simulink model "single_phase_ttype_inverter"  (R2026a)
settings: Solver=ode23tb  StopTime=simlength  FixedStep=tc  MaxStep=glb_time.tc
values from neighbouring files (symbols this model uses):
  afe_ctrl = param.afe.ctrl    [init_model.m]
  afe_pwm_phase_shift_mod1 = param.afe.behav.pwm_phase_shift_mod1    [init_model.m]
  DThs_init = param.thermal.DThs_init    [init_model.m]
  filters = param.ctrl.filters    [init_model.m]
  frt_data = param.frt.data    [init_model.m]
  glb_time = param.glb_time    [init_model.m]
  grid_emu = param.grid.emu    [init_model.m]
  kepsilon = param.spinv.kepsilon    [init_model.m]
  kp_align = param.ctrl.kp_align    [init_model.m]
  lim_down_align = param.ctrl.lim_down_align    [init_model.m]
  lim_up_align = param.ctrl.lim_up_align    [init_model.m]
  mavarage_filter_frequency_base_order = param.ctrl.mavarage_filter_frequency_base_order    [init_model.m]
  omega_set = param.spinv.omega_set    [init_model.m]
  single_phase_inverter_ctrl = param.spinv.ctrl    [init_model.m]
  Tambient = param.thermal.Tambient    [init_model.m]
  time_aux_power_supply_fault = param.sim.time_aux_power_supply_fault    [init_model.m]
  time_step_ref_1 = param.spinv.ref.time_step_ref_1    [init_model.m]
  time_step_ref_2 = param.spinv.ref.time_step_ref_2    [init_model.m]
  time_step_ref_3 = param.spinv.ref.time_step_ref_3    [init_model.m]
undefined symbols (not defined in the file or in its folder): delta_fht1, hwdata, ki_align, Ld_fht1, magnitude, omega_fht1, ts_inv, Vac_FS, Vdc_nom, Xbez
libraries: fl_lib x61, nesl_utility x39, moving_average_filter x11, moving_average_filter_cc x8, discrete_time_low_pass_filter x4, sl_discontinuities x3, single_phase_transformer_lib x3, linear_double_integrator_observer_ccaller x2, phase_shift_filter_ccaller x2, threephase_inductor_lib x1, dclink_for_two_levels x1, three_phase_pwm_modulator x1
(part 5 of 9)

== system single_phase_ttype_inverter/single_phase_inverter/single phase inverter control/single_phase_inverter_ctrl/single_phase_current_control/current_reference_generation ==
  mag_ref : Inport
  phase : Inport  Port=2
  Bus Creator : BusCreator  Inputs=2
  Product : Product
  Product1 : Product
  Sin : Trigonometry  Operator=cos
  Sin1 : Trigonometry
  is_ref : Outport
  id_ref : Outport  Port=2
  wires:
  Sin/1 -> Product/2
  phase/1 -> Sin1/1, Sin/1
  mag_ref/1 -> id_ref/1, Product1/1, Product/1
  Sin1/1 -> Product1/2
  Product/1 -> Bus Creator/1  "is_ref_alpha"
  Product1/1 -> Bus Creator/2  "is_ref_beta"
  Bus Creator/1 -> is_ref/1

== system single_phase_ttype_inverter/single_phase_inverter/single phase inverter control/single_phase_inverter_ctrl/single_phase_current_control/dqpi_current_controller ==
  id_ref : Inport
  Bus Creator : BusCreator  Inputs=3
  Bus Creator1 : BusCreator  Inputs=3
  Constant : Constant
  Variant Source : VariantSource  VariantControls={use_current_controller_from_ccaller_mod1 == 0, use_current_controller_from_ccaller_mod1 == 1}
  Variant Source1 : VariantSource  VariantControls={use_current_controller_from_ccaller_mod1 == 0, use_current_controller_from_ccaller_mod1 == 1}
  alphabeta2dq : Subsystem
  dq2alphabeta : Subsystem
  dq_vector_pi : Subsystem
  dq_vector_pi_ccaller : Subsystem
  dq_vector_pi_tracking : Scope  NumInputPorts=2
      settings: ActiveDisplayYMinimum=-0.073650141288039941  ActiveDisplayYMaximum=0.19925097179955883  DataLoggingVariableName=ScopeData8
  i2alphabeta : Subsystem
  virtual_alpha_beta_currents : Scope  NumInputPorts=3
      settings: ActiveDisplayYMinimum=-8.48572850227356  ActiveDisplayYMaximum=8.5032522678375244  DataLoggingVariableName=ScopeData2
  u_out : Outport
  tag scope: i_alpha=scoped, i_beta=scoped, id=scoped, id_ref=scoped, iq=scoped, ud_ctrl=scoped, uq_ctrl=scoped
  wires:
  dq2alphabeta/1(alpha) -> u_out/1
  id_ref/1 -> dq_vector_pi/1(id_ref), Bus Creator/1, [id_ref], dq_vector_pi_ccaller/2(id_ref)
  alphabeta2dq/1("d ") -> Bus Creator/2, [id], dq_vector_pi_ccaller/1(id), dq_vector_pi/2(id)  "id"
  alphabeta2dq/2("q ") -> dq_vector_pi/3(iq), Bus Creator1/2, [iq], dq_vector_pi_ccaller/3(iq)  "iq"
  [iq_ref] -> dq_vector_pi/4(iq_ref), dq_vector_pi_ccaller/4(iq_ref)
  Variant Source1/1 -> dq2alphabeta/2(q)  "ctrl_q_u"
  Variant Source/1 -> dq2alphabeta/1(d)  "ctrl_d_u"
  dq_vector_pi/1(ud_ctrl) -> Variant Source/1
  dq_vector_pi/2(uq_ctrl) -> Variant Source1/1
  Constant/1 -> dq_vector_pi_ccaller/5(udc_pu)
  dq_vector_pi_ccaller/1(ud_ctrl_out) -> [ud_ctrl], Variant Source/2
  dq_vector_pi_ccaller/2(uq_ctrl_out) -> [uq_ctrl], Variant Source1/2
  Bus Creator1/1 -> dq_vector_pi_tracking/2
  Bus Creator/1 -> dq_vector_pi_tracking/1
  [ud_ctrl] -> Bus Creator/3
  [uq_ctrl] -> Bus Creator1/3
  [iq_ref] -> Bus Creator1/1
  [inverter_current_output_pu] -> i2alphabeta/1(i_alpha), virtual_alpha_beta_currents/1  "i_load"
  i2alphabeta/1(i_alpha_out) -> alphabeta2dq/1(alpha), virtual_alpha_beta_currents/2, [i_alpha]  "i_alpha"
  i2alphabeta/2(i_beta_out) -> alphabeta2dq/2(beta), virtual_alpha_beta_currents/3, [i_beta]  "i_beta"

== system single_phase_ttype_inverter/single_phase_inverter/single phase inverter control/single_phase_inverter_ctrl/single_phase_current_control/rpi_current_controller ==
  i_ref : Inport
  Bus Creator : BusCreator  Inputs=3
  Bus Selector : BusSelector  OutputSignals=u_out
  Bus Selector1 : BusSelector  OutputSignals=is_ref_alpha
  C Caller : CCaller  FunctionName=rpi_process_simulink  PortSpecificationStruct="%)30     .    V!(   8    (     @         %    \"     L    !     0         %  0 \"0    $    _    07)G3F%M90  4&]R=$YA;64 4V-O<&4     26YD97@     5'EP90      4VEZ90      27-';&]B86P   X    P    !@    @    $          4    (     0    ,    !         !   P!O=70 #@   #     &    \"     0         !0    @    !     P    $         $  # &]U=  .    .     8    (    !          %    \"     $    &     0         0   ...(+6126 chars)"
  Constant : Constant  Value=single_phase_inverter_ctrl.ki_rpi
  Constant1 : Constant  Value=omega_set
  Constant2 : Constant  Value=single_phase_inverter_ctrl.delta_rpi
  Constant3 : Constant  Value=glb_time.ts_inv
  Constant4 : Constant
  Constant5 : Constant  Value=single_phase_inverter_ctrl.kp_rpi
  Data Type Conversion{,1..2,4..6,9..10,13} (9 alike) : DataTypeConversion  OutDataTypeStr=single  SaturateOnIntegerOverflow=off  RndMeth=Floor
  Data Type Conversion7 : DataTypeConversion  OutDataTypeStr=double  SaturateOnIntegerOverflow=off  RndMeth=Floor
  Data Type Conversion8 : DataTypeConversion  OutDataTypeStr=uint8  SaturateOnIntegerOverflow=off  RndMeth=Floor
  Reset : Subsystem
  rpi_tracking : Scope
      settings: ActiveDisplayYMinimum=-0.4355491582306612  ActiveDisplayYMaximum=0.450079712585125  DataLoggingVariableName=ScopeData14
  u_ctrl_out : Outport
  tag scope: rpi_tracking_i=scoped, rpi_tracking_iref=scoped, rpi_tracking_uout=scoped
  wires:
  Constant4/1 -> Data Type Conversion13/1
  Constant2/1 -> Data Type Conversion10/1
  Constant1/1 -> Data Type Conversion9/1
  Constant/1 -> Data Type Conversion6/1
  Data Type Conversion8/1 -> C Caller/1
  Data Type Conversion/1 -> C Caller/2
  Data Type Conversion1/1 -> C Caller/3
  Data Type Conversion2/1 -> C Caller/4
  Data Type Conversion4/1 -> C Caller/5
  Data Type Conversion5/1 -> C Caller/6
  Data Type Conversion6/1 -> C Caller/7
  Data Type Conversion9/1 -> C Caller/8
  Data Type Conversion10/1 -> C Caller/9
  Data Type Conversion13/1 -> C Caller/10
  Constant3/1 -> Data Type Conversion4/1
  Constant5/1 -> Data Type Conversion5/1
  [dclink_voltage_pu] -> Data Type Conversion2/1
  [inverter_current_output_pu] -> [rpi_tracking_i], Bus Creator/2, Data Type Conversion1/1
  i_ref/1 -> Bus Selector1/1
  Reset/1(en) -> Data Type Conversion8/1
  C Caller/1 -> Bus Selector/1  "out"
  Bus Selector/1 -> Data Type Conversion7/1  "<u_out>"
  Bus Selector1/1 -> [rpi_tracking_iref], Bus Creator/1, Data Type Conversion/1  "<is_ref_alpha>"
  Bus Creator/1 -> rpi_tracking/1
  Data Type Conversion7/1 -> u_ctrl_out/1, [rpi_tracking_uout], Bus Creator/3  "u_ctrl_out"

== system single_phase_ttype_inverter/single_phase_inverter/single phase inverter control/single_phase_inverter_ctrl/sistem_identification/open loop u//f ==
  Constant2 : Constant  Value=0.75
  Data Store Memory : DataStoreMemory  DataStoreName=u_test  WriteAfterWriteMsg=warning  ShowAdditionalParam=off
  Data Store Read1 : DataStoreRead  DataStoreName=u_test  DataStoreElements=u_test  IndexOptions=Index vector (dialog)  Indices=1  OutputSizes=1
  Data Store Write : DataStoreWrite  DataStoreName=u_test  IndexOptions=Index vector (dialog)  Indices=1  OutputSizes=1
  Gain1 : Gain  Gain=1/omega_set
  Gain2 : Gain  Gain=Vdc_nom/Vac_FS
  Gain3 : Gain  Gain=Xbez
  Product : Product  Inputs=*/
  Saturation : Saturate  UpperLimit=inf  LowerLimit=0.1
  dq2alphabeta : Subsystem
  first_harmonic_tracker : Subsystem  Commented=on
  i_alpha_beta_system_identification : Scope  NumInputPorts=4
      settings: ActiveDisplayYMinimum=1.5097956747477865  ActiveDisplayYMaximum=1.9442466663089897  DataLoggingVariableName=ScopeData2
  module : Subsystem
  phase_shift_filter_ccaller : phase_shift_filter_ccaller/phase_shift_filter_ccaller  Commented=on  freq_m=frequency_set  ts_m=ts_inv  scaling_m=phase_shift_filter_gain  reset_time_release=0.025  instance=1  tc_m=-1
  sogi_ccaller : Subsystem
  u_out : Outport
  tag scope: impedance_load_estimator=scoped, load_inductance_estimated=scoped
  wires:
  [inverter_current_output_pu] -> sogi_ccaller/1(input)  "i_alpha"
  dq2alphabeta/1(alpha) -> u_out/1
  Data Store Read1/1 -> Product/1
  Constant2/1 -> Data Store Write/1
  Saturation/1 -> Product/2
  module/1(i) -> Saturation/1  "Iload"
  Product/1 -> Gain2/1
  Gain1/1 -> [load_inductance_estimated], i_alpha_beta_system_identification/2  "Lload"
  sogi_ccaller/1(alpha) -> i_alpha_beta_system_identification/3, module/1(i_alpha)  "i_alpha_sogi"
  sogi_ccaller/2(beta) -> i_alpha_beta_system_identification/4, module/2(i_beta)  "i_beta_sogi"
  Gain2/1 -> Gain3/1
  Gain3/1 -> [impedance_load_estimator], i_alpha_beta_system_identification/1, Gain1/1  "Xload"

== system single_phase_ttype_inverter/afe/AFE_control/afe_control/FRT-VDE4110/FRT-Detection/voltage_rate_measure_neg ==
  v_grid_neg_xi_avg : Inport
  Abs1 : Abs  SaturateOnIntegerOverflow=off
  linear_double_integrator_observer_ccaller : linear_double_integrator_observer_ccaller/linear_double_integrator_observer_ccaller  kx_m=afe_ctrl.vr_obs.kx  kv_m=afe_ctrl.vr_obs.kv  ts_m=glb_time.ts_afe  time_release=0.025  instance=0  tc_m=-1
  vxi_neg_dot : Outport
  wires:
  linear_double_integrator_observer_ccaller/2 -> Abs1/1
  v_grid_neg_xi_avg/1 -> linear_double_integrator_observer_ccaller/1
  Abs1/1 -> vxi_neg_dot/1  "vxi_neg_dot"

== system single_phase_ttype_inverter/afe/AFE_control/afe_control/FRT-VDE4110/FRT-Detection/voltage_rate_measure_pos ==
  v_grid_pos_xi_avg : Inport
  Abs : Abs  SaturateOnIntegerOverflow=off
  linear_double_integrator_observer_ccaller : linear_double_integrator_observer_ccaller/linear_double_integrator_observer_ccaller  kx_m=afe_ctrl.vr_obs.kx  kv_m=afe_ctrl.vr_obs.kv  ts_m=glb_time.ts_afe  time_release=0.025  instance=0  tc_m=-1
  vxi_pos_dot : Outport
  wires:
  linear_double_integrator_observer_ccaller/2 -> Abs/1
  Abs/1 -> vxi_pos_dot/1  "vxi_pos_dot"
  v_grid_pos_xi_avg/1 -> linear_double_integrator_observer_ccaller/1

== system single_phase_ttype_inverter/afe/AFE_control/afe_control/FRT-VDE4110/FRT-PosNegReactiveCurrentReferences/avg_flt_500ms ==
  In1 : Inport
  Constant : Constant  Value=2*pi/500e-3
  Constant1 : Constant  Value=glb_time.ts_afe
  Constant2 : Constant
  Sum : Sum  Inputs=|-+
  avg_flt_1 : MATLAB Function  TreatAsAtomicUnit=on
  Out1 : Outport  VectorParamsAs1DForOutWhenUnconnected=off
  wires:
  avg_flt_1/1(y1) -> Out1/1  "output"
  Constant1/1 -> avg_flt_1/3(ts)
  Constant/1 -> avg_flt_1/2(w)
  In1/1 -> avg_flt_1/1(x)  "input"
  Constant2/1 -> Sum/2
  [frt_active_mod1] -> Sum/1
  Sum/1 -> avg_flt_1/4(enable)

== system single_phase_ttype_inverter/afe/AFE_control/afe_control/FRT-VDE4110/FRT-PosNegReactiveCurrentReferences/avg_flt_500ms1 ==
  In1 : Inport
  Constant : Constant  Value=2*pi/500e-3
  Constant1 : Constant  Value=glb_time.ts_afe
  Constant2 : Constant
  Sum : Sum  Inputs=|-+
  avg_flt_1 : MATLAB Function  TreatAsAtomicUnit=on
  Out1 : Outport  VectorParamsAs1DForOutWhenUnconnected=off
  wires:
  Sum/1 -> avg_flt_1/4(enable)
  [frt_active_mod1] -> Sum/1
  Constant2/1 -> Sum/2
  In1/1 -> avg_flt_1/1(x)  "input"
  Constant/1 -> avg_flt_1/2(w)
  Constant1/1 -> avg_flt_1/3(ts)
  avg_flt_1/1(y1) -> Out1/1  "output"

== system single_phase_ttype_inverter/afe/AFE_control/afe_control/FRT-VDE4110/FRT-PosNegReactiveCurrentReferences/avg_flt_500ms2 ==
  In1 : Inport
  Constant : Constant  Value=2*pi/500e-3
  Constant1 : Constant  Value=glb_time.ts_afe
  Constant2 : Constant
  Sum : Sum  Inputs=|-+
  avg_flt_1 : MATLAB Function  TreatAsAtomicUnit=on
  Out1 : Outport  VectorParamsAs1DForOutWhenUnconnected=off
  wires:
  avg_flt_1/1(y1) -> Out1/1  "output"
  Constant1/1 -> avg_flt_1/3(ts)
  Constant/1 -> avg_flt_1/2(w)
  In1/1 -> avg_flt_1/1(x)  "input"
  Constant2/1 -> Sum/2
  [frt_active_mod1] -> Sum/1
  Sum/1 -> avg_flt_1/4(enable)

== system single_phase_ttype_inverter/afe/AFE_control/afe_control/FRT-VDE4110/FRT-PosNegReactiveCurrentReferences/avg_flt_500ms3 ==
  In1 : Inport
  Constant : Constant  Value=2*pi/500e-3
  Constant1 : Constant  Value=glb_time.ts_afe
  Constant2 : Constant
  Sum : Sum  Inputs=|-+
  avg_flt_1 : MATLAB Function  TreatAsAtomicUnit=on
  Out1 : Outport  VectorParamsAs1DForOutWhenUnconnected=off
  wires:
  Sum/1 -> avg_flt_1/4(enable)
  [frt_active_mod1] -> Sum/1
  Constant2/1 -> Sum/2
  In1/1 -> avg_flt_1/1(x)  "input"
  Constant/1 -> avg_flt_1/2(w)
  Constant1/1 -> avg_flt_1/3(ts)
  avg_flt_1/1(y1) -> Out1/1  "output"

== system single_phase_ttype_inverter/afe/AFE_control/afe_control/FRT-VDE4110/FRT-PosNegReactiveCurrentReferences/u_161Hz_flt1 ==
  input : Inport
  Gain3 : Gain  Gain=filters.afe.g1_161Hz
  Gain6 : Gain  Gain=filters.afe.g0_161Hz
  Sum : Sum  Inputs=|++
  Unit Delay1 : UnitDelay  SampleTime=-1
  output : Outport  VectorParamsAs1DForOutWhenUnconnected=off
  wires:
  Gain6/1 -> Sum/1
  input/1 -> Gain6/1
  Unit Delay1/1 -> Gain3/1
  Gain3/1 -> Sum/2
  Sum/1 -> Unit Delay1/1, output/1

== system single_phase_ttype_inverter/afe/AFE_control/afe_control/FRT-VDE4110/FRT-PosNegReactiveCurrentReferences/u_161Hz_flt2 ==
  input : Inport
  Gain3 : Gain  Gain=filters.afe.g1_161Hz
  Gain6 : Gain  Gain=filters.afe.g0_161Hz
  Sum : Sum  Inputs=|++
  Unit Delay1 : UnitDelay  SampleTime=-1
  output : Outport  VectorParamsAs1DForOutWhenUnconnected=off
  wires:
  Sum/1 -> output/1, Unit Delay1/1
  Gain3/1 -> Sum/2
  Unit Delay1/1 -> Gain3/1
  input/1 -> Gain6/1
  Gain6/1 -> Sum/1

== system single_phase_ttype_inverter/afe/AFE_control/afe_control/FRT-VDE4110/FRT-PosNegReactiveCurrentReferences/u_161Hz_flt3 ==
  input : Inport
  Gain3 : Gain  Gain=filters.afe.g1_161Hz
  Gain6 : Gain  Gain=filters.afe.g0_161Hz
  Sum : Sum  Inputs=|++
  Unit Delay1 : UnitDelay  SampleTime=-1
  output : Outport  VectorParamsAs1DForOutWhenUnconnected=off
  wires:
  Gain6/1 -> Sum/1
  input/1 -> Gain6/1
  Unit Delay1/1 -> Gain3/1
  Gain3/1 -> Sum/2
  Sum/1 -> Unit Delay1/1, output/1

== system single_phase_ttype_inverter/afe/AFE_control/afe_control/current_ctrl/inner_current_ctrl/anti_wind_up_ff ==
  d_abc : Inport
  Add : Sum
  Bus Creator : BusCreator  Inputs=3
  Bus Creator1 : BusCreator  Inputs=2
  Demux1 : Demux  Outputs=3
  MATLAB Function : MATLAB Function  TreatAsAtomicUnit=on
  MATLAB Function1 : MATLAB Function  TreatAsAtomicUnit=on
  Unit Delay1 : UnitDelay  SampleTime=-1
  Unit Delay2 : UnitDelay  SampleTime=-1
  Unit Delay3 : UnitDelay  SampleTime=-1
  afe_ictrl_out/afe_ictrl_ff : Scope  NumInputPorts=3
      settings: ActiveDisplayYMinimum=-2.3644997050526393  ActiveDisplayYMaximum=2.3332899605671109  DataLoggingVariableName=ScopeData4
  anti_wind_up : Subsystem
  u_ctrl_out : Outport
  wires:
  d_abc/1 -> Add/1, afe_ictrl_out/afe_ictrl_ff/2  "d_abc"
  Add/1 -> Demux1/1  "d_abc_sum"
  Unit Delay3/1 -> anti_wind_up/2(beta), Bus Creator1/2  "ubeta_afe"
  Unit Delay1/1 -> afe_ictrl_out/afe_ictrl_ff/3  "u_grid_ff_abc_mod1"
  Unit Delay2/1 -> Bus Creator1/1, anti_wind_up/1(alpha)  "ualpha_afe"
  MATLAB Function/2(beta) -> Unit Delay3/1  "u_beta"
  [v_grid_ff_abc_mod1] -> Unit Delay1/1
  Bus Creator1/1 -> u_ctrl_out/1
  MATLAB Function/1(alpha) -> Unit Delay2/1  "u_alpha"
  anti_wind_up/1(scaling) -> MATLAB Function1/4(scaling)
  MATLAB Function1/1(das) -> Bus Creator/1, MATLAB Function/1(a)  "das"
  MATLAB Function1/2(dbs) -> Bus Creator/2, MATLAB Function/2(b)  "dbs"
  MATLAB Function1/3(dcs) -> Bus Creator/3, MATLAB Function/3(c)  "dcs"
  Demux1/3 -> MATLAB Function1/3(dc)  "dc"
  Demux1/2 -> MATLAB Function1/2(db)  "db"
  Demux1/1 -> MATLAB Function1/1(da)  "da"
  Bus Creator/1 -> afe_ictrl_out/afe_ictrl_ff/1  "ds_abc"

== system single_phase_ttype_inverter/afe/AFE_control/afe_control/current_ctrl/inner_current_ctrl/rpi_phase_a ==
  In1 : Inport
  In2 : Inport  Port=2
  Add : Sum
  Cresd : Gain  Gain=afe_ctrl.res_pi.Cresd  Multiplication=Matrix(K*u)
  Gain : Gain  Gain=afe_ctrl.res_pi.kp_rpi
  Gain1 : Gain  Gain=afe_ctrl.res_pi.ki_rpi
  Gain2 : Gain  Gain=afe_ctrl.res_pi.Bresd  Multiplication=Matrix(K*u)
  Gain3 : Gain  Gain=afe_ctrl.res_pi.Aresd  Multiplication=Matrix(K*u)
  Sum : Sum  Inputs=|+-
  Sum2 : Sum  Inputs=|++  SaturateOnIntegerOverflow=on
  Unit Delay : UnitDelay  InitialCondition=[0 0]  SampleTime=-1
  Out1 : Outport
  wires:
  In1/1 -> Sum/1  "isa_ref"
  In2/1 -> Sum/2  "isa"
  Add/1 -> Out1/1  "da"
  Sum/1 -> Gain1/1, Gain/1
  Gain/1 -> Add/1
  Gain1/1 -> Gain2/1  "u(k)"
  Gain2/1 -> Sum2/1
  Unit Delay/1 -> Gain3/1, Cresd/1  "x(k)"
  Sum2/1 -> Unit Delay/1  "x(k+1)"
  Gain3/1 -> Sum2/2
  Cresd/1 -> Add/2  "y(k)"

== system single_phase_ttype_inverter/afe/AFE_control/afe_control/current_ctrl/inner_current_ctrl/rpi_phase_b ==
  In1 : Inport
  In2 : Inport  Port=2
  Add : Sum
  Cresd : Gain  Gain=afe_ctrl.res_pi.Cresd  Multiplication=Matrix(K*u)
  Gain : Gain  Gain=afe_ctrl.res_pi.kp_rpi
  Gain1 : Gain  Gain=afe_ctrl.res_pi.ki_rpi
  Gain2 : Gain  Gain=afe_ctrl.res_pi.Bresd  Multiplication=Matrix(K*u)
  Gain3 : Gain  Gain=afe_ctrl.res_pi.Aresd  Multiplication=Matrix(K*u)
  Sum : Sum  Inputs=|+-
  Sum2 : Sum  Inputs=|++  SaturateOnIntegerOverflow=on
  Unit Delay : UnitDelay  InitialCondition=[0 0]  SampleTime=-1
  Out1 : Outport
  wires:
  Cresd/1 -> Add/2  "y(k)"
  Gain3/1 -> Sum2/2
  Sum2/1 -> Unit Delay/1  "x(k+1)"
  Unit Delay/1 -> Cresd/1, Gain3/1  "x(k)"
  Gain2/1 -> Sum2/1
  Gain1/1 -> Gain2/1  "u(k)"
  Gain/1 -> Add/1
  Sum/1 -> Gain/1, Gain1/1
  Add/1 -> Out1/1  "da"
  In2/1 -> Sum/2  "isa"
  In1/1 -> Sum/1  "isa_ref"

== system single_phase_ttype_inverter/afe/AFE_control/afe_control/current_ctrl/inner_current_ctrl/rpi_phase_c ==
  In1 : Inport
  In2 : Inport  Port=2
  Add : Sum
  Cresd : Gain  Gain=afe_ctrl.res_pi.Cresd  Multiplication=Matrix(K*u)
  Gain : Gain  Gain=afe_ctrl.res_pi.kp_rpi
  Gain1 : Gain  Gain=afe_ctrl.res_pi.ki_rpi
  Gain2 : Gain  Gain=afe_ctrl.res_pi.Bresd  Multiplication=Matrix(K*u)
  Gain3 : Gain  Gain=afe_ctrl.res_pi.Aresd  Multiplication=Matrix(K*u)
  Sum : Sum  Inputs=|+-
  Sum2 : Sum  Inputs=|++  SaturateOnIntegerOverflow=on
  Unit Delay : UnitDelay  InitialCondition=[0 0]  SampleTime=-1
  Out1 : Outport
  wires:
  In1/1 -> Sum/1  "isa_ref"
  In2/1 -> Sum/2  "isa"
  Add/1 -> Out1/1  "da"
  Sum/1 -> Gain1/1, Gain/1
  Gain/1 -> Add/1
  Gain1/1 -> Gain2/1  "u(k)"
  Gain2/1 -> Sum2/1
  Unit Delay/1 -> Gain3/1, Cresd/1  "x(k)"
  Sum2/1 -> Unit Delay/1  "x(k+1)"
  Gain3/1 -> Sum2/2
  Cresd/1 -> Add/2  "y(k)"

== system single_phase_ttype_inverter/afe/AFE_control/afe_control/grid_current_sequences_and_reactive_pwr_ctrl/current_sequence_avg/average_filter ==
  i_grid_pos_xi : Inport
  i_grid_pos_eta : Inport  Port=2
  i_grid_neg_xi : Inport  Port=3
  i_grid_neg_eta : Inport  Port=4
  Abs : Abs  SaturateOnIntegerOverflow=off
  Gain : Gain  Gain=grid_emu.omega_grid_nom*mavarage_filter_frequency_base_order
  Saturation : Saturate  UpperLimit=2  LowerLimit=0.1
  dmavg_flt{,1..3} (4 alike) : moving_average_filter/dmavg_flt  ts=glb_time.ts_afe  enable_time=dmavg_filter_enable_time
  i_grid_pos_xi_avg : Outport
  i_grid_pos_eta_avg : Outport  Port=2
  i_grid_neg_xi_avg : Outport  Port=3
  i_grid_neg_eta_avg : Outport  Port=4
  wires:
  i_grid_pos_eta/1 -> dmavg_flt1/1
  Gain/1 -> dmavg_flt/2, dmavg_flt1/2, dmavg_flt3/2, dmavg_flt2/2
  dmavg_flt/1 -> i_grid_pos_xi_avg/1
  i_grid_neg_eta/1 -> dmavg_flt3/1
  i_grid_pos_xi/1 -> dmavg_flt/1
  dmavg_flt2/1 -> i_grid_neg_xi_avg/1
  i_grid_neg_xi/1 -> dmavg_flt2/1
  dmavg_flt3/1 -> i_grid_neg_eta_avg/1
  dmavg_flt1/1 -> i_grid_pos_eta_avg/1
  Abs/1 -> Saturation/1
  Saturation/1 -> Gain/1
  [omega_grid_pll_pu_mod1] -> Abs/1

== system single_phase_ttype_inverter/afe/AFE_control/afe_control/grid_current_sequences_and_reactive_pwr_ctrl/current_sequence_avg/average_filter_ccaller ==
  i_grid_pos_xi : Inport
  i_grid_pos_eta : Inport  Port=2
  i_grid_neg_xi : Inport  Port=3
  i_grid_neg_eta : Inport  Port=4
  Abs : Abs  SaturateOnIntegerOverflow=off
  Gain : Gain  Gain=grid_emu.omega_grid_nom*mavarage_filter_frequency_base_order
  Saturation : Saturate  UpperLimit=2  LowerLimit=0.1
  dmavg_flt : moving_average_filter_cc/dmavg_flt  instance=4  ts=glb_time.ts_afe  enable_time=dmavg_filter_enable_time
  dmavg_flt1 : moving_average_filter_cc/dmavg_flt  instance=5  ts=glb_time.ts_afe  enable_time=dmavg_filter_enable_time
  dmavg_flt2 : moving_average_filter_cc/dmavg_flt  instance=6  ts=glb_time.ts_afe  enable_time=dmavg_filter_enable_time
  dmavg_flt3 : moving_average_filter_cc/dmavg_flt  instance=7  ts=glb_time.ts_afe  enable_time=dmavg_filter_enable_time
  i_grid_pos_xi_avg : Outport
  i_grid_pos_eta_avg : Outport  Port=2
  i_grid_neg_xi_avg : Outport  Port=3
  i_grid_neg_eta_avg : Outport  Port=4
  wires:
  dmavg_flt1/1 -> i_grid_pos_eta_avg/1
  dmavg_flt3/1 -> i_grid_neg_eta_avg/1
  i_grid_neg_xi/1 -> dmavg_flt2/1
  dmavg_flt2/1 -> i_grid_neg_xi_avg/1
  i_grid_pos_xi/1 -> dmavg_flt/1
  i_grid_neg_eta/1 -> dmavg_flt3/1
  dmavg_flt/1 -> i_grid_pos_xi_avg/1
  Gain/1 -> dmavg_flt/2, dmavg_flt1/2, dmavg_flt3/2, dmavg_flt2/2
  i_grid_pos_eta/1 -> dmavg_flt1/1
  Abs/1 -> Saturation/1
  Saturation/1 -> Gain/1
  [omega_grid_pll_pu_mod1] -> Abs/1

== system single_phase_ttype_inverter/afe/AFE_control/afe_control/grid_current_sequences_and_reactive_pwr_ctrl/sequences_current_control/Negative-Seq. eta-Control ==
  ff : Inport
  e : Inport  Port=2
  1/Ti : Gain  Gain=afe_ctrl.kp_rc_neg_grid  SaturateOnIntegerOverflow=on  OutDataTypeStr=Inherit: Same as input  ParamDataTypeStr=Inherit: Same as input
  Saturation : Saturate  UpperLimit=afe_ctrl.ieta_neg_ref_lim  LowerLimit=-afe_ctrl.ieta_neg_ref_lim
  Sum : Sum  Inputs=|++
  Sum2 : Sum  Inputs=+++  SaturateOnIntegerOverflow=on
  Sum3 : Sum  Inputs=-+  SaturateOnIntegerOverflow=on
  Unit Delay4 : UnitDelay  SampleTime=-1
  kp : Gain  Gain=afe_ctrl.ki_rc_neg_grid*glb_time.ts_afe  SaturateOnIntegerOverflow=on  OutDataTypeStr=Inherit: Same as input  ParamDataTypeStr=Inherit: Same as input
  u : Outport  VectorParamsAs1DForOutWhenUnconnected=off
  wires:
  Unit Delay4/1 -> Sum2/3
  Sum3/1 -> Unit Delay4/1
  kp/1 -> Sum2/2
  Sum2/1 -> Saturation/1
  1/Ti/1 -> Sum2/1, Sum3/1
  Saturation/1 -> Sum/1, Sum3/2
  Sum/1 -> u/1
  e/1 -> 1/Ti/1, kp/1  "e"
  ff/1 -> Sum/2

== system single_phase_ttype_inverter/afe/AFE_control/afe_control/grid_current_sequences_and_reactive_pwr_ctrl/sequences_current_control/Negative-Seq. xi-Control ==
  ff : Inport
  e : Inport  Port=2
  1/Ti : Gain  Gain=afe_ctrl.kp_rc_neg_grid  SaturateOnIntegerOverflow=on  OutDataTypeStr=Inherit: Same as input  ParamDataTypeStr=Inherit: Same as input
  Saturation : Saturate  UpperLimit=afe_ctrl.ieta_pos_ref_lim  LowerLimit=-afe_ctrl.ieta_pos_ref_lim
  Sum : Sum  Inputs=|++
  Sum2 : Sum  Inputs=+++  SaturateOnIntegerOverflow=on
  Sum3 : Sum  Inputs=-+  SaturateOnIntegerOverflow=on
  Unit Delay4 : UnitDelay  SampleTime=-1
  kp : Gain  Gain=afe_ctrl.ki_rc_neg_grid*glb_time.ts_afe  SaturateOnIntegerOverflow=on  OutDataTypeStr=Inherit: Same as input  ParamDataTypeStr=Inherit: Same as input
  u : Outport  VectorParamsAs1DForOutWhenUnconnected=off
  wires:
  Unit Delay4/1 -> Sum2/3
  Sum3/1 -> Unit Delay4/1
  kp/1 -> Sum2/2
  Sum2/1 -> Saturation/1
  1/Ti/1 -> Sum2/1, Sum3/1
  Saturation/1 -> Sum/1, Sum3/2
  Sum/1 -> u/1
  e/1 -> 1/Ti/1, kp/1  "e"
  ff/1 -> Sum/2

== system single_phase_ttype_inverter/afe/AFE_control/afe_control/grid_current_sequences_and_reactive_pwr_ctrl/sequences_current_control/Positive-Seq. eta-Control ==
  ff : Inport
  e : Inport  Port=2
  1/Ti : Gain  Gain=afe_ctrl.kp_rc_pos_grid  SaturateOnIntegerOverflow=on  OutDataTypeStr=Inherit: Same as input  ParamDataTypeStr=Inherit: Same as input
  Saturation : Saturate  UpperLimit=afe_ctrl.ieta_pos_ref_lim  LowerLimit=-afe_ctrl.ieta_pos_ref_lim
  Sum : Sum  Inputs=|++
  Sum2 : Sum  Inputs=+++  SaturateOnIntegerOverflow=on
  Sum3 : Sum  Inputs=-+  SaturateOnIntegerOverflow=on
  Unit Delay4 : UnitDelay  SampleTime=-1
  kp : Gain  Gain=afe_ctrl.ki_rc_pos_grid*glb_time.ts_afe  SaturateOnIntegerOverflow=on  OutDataTypeStr=Inherit: Same as input  ParamDataTypeStr=Inherit: Same as input
  u : Outport  VectorParamsAs1DForOutWhenUnconnected=off
  wires:
  Unit Delay4/1 -> Sum2/3
  Sum3/1 -> Unit Delay4/1
  kp/1 -> Sum2/2
  Sum2/1 -> Saturation/1
  1/Ti/1 -> Sum2/1, Sum3/1
  Saturation/1 -> Sum/1, Sum3/2
  Sum/1 -> u/1
  e/1 -> 1/Ti/1, kp/1  "e"
  ff/1 -> Sum/2

== system single_phase_ttype_inverter/afe/AFE_control/afe_control/grid_voltage_phase_lock_loops/DDSRF-PLL/pll_stageA ==
  gamma_grid : Inport
  ug_abc_pu : Inport  Port=2
  Demux : Demux  Outputs=3
  Math Function : Math  Operator=magnitude^2  SignedPower=on
  Math Function1 : Math  Operator=magnitude^2  SignedPower=on
  Reciprocal Sqrt : Sqrt  Operator=rSqrt
  Saturation : Saturate  UpperLimit=inf  LowerLimit=0.02
  Sum : Sum  Inputs=|++
  filter_and_transformation : Subsystem
  sequences : Subsystem
  u_grid_pos_xi : Outport  VectorParamsAs1DForOutWhenUnconnected=off
  u_grid_pos_eta : Outport  Port=2  VectorParamsAs1DForOutWhenUnconnected=off
  tag scope: Vgrid_unorm_ddsrf=scoped
  wires:
  Saturation/1 -> Reciprocal Sqrt/1
  Reciprocal Sqrt/1 -> [Vgrid_unorm_ddsrf]
  Sum/1 -> Saturation/1
  Math Function1/1 -> Sum/2
  Math Function/1 -> Sum/1
  filter_and_transformation/2(ug_beta) -> Math Function1/1, sequences/2(u_grid_beta)
  filter_and_transformation/1(ug_alpha) -> Math Function/1, sequences/1(u_grid_alpha)
  Demux/3 -> filter_and_transformation/3(ug_c)
  Demux/2 -> filter_and_transformation/2(ug_b)
  Demux/1 -> filter_and_transformation/1(ug_a)
  ug_abc_pu/1 -> Demux/1
  sequences/1(u_grid_pos_xi) -> u_grid_pos_xi/1
  sequences/2(u_grid_pos_eta) -> u_grid_pos_eta/1
  gamma_grid/1 -> sequences/3(phase_angle)

== system single_phase_ttype_inverter/afe/AFE_control/afe_control/grid_voltage_phase_lock_loops/DDSRF-PLL/pll_stageB ==
  u_grid_pos_xi : Inport
  u_grid_pos_eta : Inport  Port=2
  Constant4 : Constant  Value=grid_emu.omega_grid_nom
  Gain : Gain  Gain=-1
  Product : Product  RndMeth=Zero
  Product1 : Product  RndMeth=Zero
  Product2 : Product  RndMeth=Zero
  Sum3 : Sum  SaturateOnIntegerOverflow=on
  Sum4 : Sum  SaturateOnIntegerOverflow=on
  Sum5 : Sum  Inputs=++|
  Terminator : Terminator
  To Workspace5 : ToWorkspace  VariableName=vgrid_xi_pll_pos  SampleTime=-1
      settings: MaxDataPoints=glb_time.Ns_afe
  To Workspace6 : ToWorkspace  VariableName=vgrid_eta_pll_pos  SampleTime=-1
      settings: MaxDataPoints=glb_time.Ns_afe
  Unit Delay1 : UnitDelay  SampleTime=-1
  Unit Delay2 : UnitDelay  SampleTime=-1
  Unit Delay4 : UnitDelay  SampleTime=-1
  bounder1 : MATLAB Function  TreatAsAtomicUnit=on
  double_integrator_observer : Subsystem
  kp : Gain  Gain=afe_ctrl.pll_i1_ddsrt*glb_time.ts_afe  SaturateOnIntegerOverflow=on  OutDataTypeStr=Inherit: Same as input  ParamDataTypeStr=Inherit: Same as input
  kp1 : Gain  Gain=afe_ctrl.pll_p_ddsrt  SaturateOnIntegerOverflow=on  OutDataTypeStr=Inherit: Same as input  ParamDataTypeStr=Inherit: Same as input
  kp2 : Gain  Gain=glb_time.ts_afe  SaturateOnIntegerOverflow=on  OutDataTypeStr=Inherit: Same as input  ParamDataTypeStr=Inherit: Same as input
  kp3 : Gain  Gain=1/grid_emu.omega_grid_nom  SaturateOnIntegerOverflow=on  OutDataTypeStr=Inherit: Same as input  ParamDataTypeStr=Inherit: Same as input
  phase_grid_ddsrf_pll : Outport  VectorParamsAs1DForOutWhenUnconnected=off
  omega_grid_ddsrf_pll : Outport  Port=2  VectorParamsAs1DForOutWhenUnconnected=off
  wires:
  Unit Delay2/1 -> double_integrator_observer/1(phase), phase_grid_ddsrf_pll/1
  kp1/1 -> Sum5/1
  Product2/1 -> kp2/1
  u_grid_pos_eta/1 -> Product1/1, To Workspace6/1
  u_grid_pos_xi/1 -> To Workspace5/1, Product/1
  bounder1/1(y) -> Unit Delay1/1, Unit Delay2/1
  Sum5/1 -> Product2/1
  kp/1 -> Sum3/1
  [Vgrid_unorm_ddsrf] -> Product1/2, Product/2
  Constant4/1 -> Product2/2
  kp2/1 -> Sum4/1
  Sum3/1 -> Unit Delay4/1, Sum5/2  "i1"
  Unit Delay1/1 -> Sum4/2
  Sum4/1 -> bounder1/1(u)
  Unit Delay4/1 -> Sum3/2
  double_integrator_observer/1(omega_hat) -> kp3/1
  Product/1 -> Terminator/1
  kp3/1 -> omega_grid_ddsrf_pll/1
  Product1/1 -> Gain/1
  Gain/1 -> kp1/1, kp/1

== system single_phase_ttype_inverter/afe/AFE_control/afe_control/grid_voltage_phase_lock_loops/FHT-PLL/pll_stageA ==
  gamma_grid : Inport
  ug_abc_pu : Inport  Port=2
  Demux : Demux  Outputs=3
  Math Function : Math  Operator=magnitude^2  SignedPower=on
  Math Function1 : Math  Operator=magnitude^2  SignedPower=on
  Reciprocal Sqrt : Sqrt  Operator=rSqrt
  Saturation : Saturate  UpperLimit=inf  LowerLimit=0.02
  Sum : Sum  Inputs=|++
  filter_and_transformation : Subsystem
  sequences : Subsystem
  u_grid_xi : Outport  VectorParamsAs1DForOutWhenUnconnected=off
  u_grid_eta : Outport  Port=2  VectorParamsAs1DForOutWhenUnconnected=off
  tag scope: Vgrid_unorm_fht=scoped
  wires:
  gamma_grid/1 -> sequences/3(phase_angle)
  sequences/2(u_grid_eta) -> u_grid_eta/1
  sequences/1(u_grid_xi) -> u_grid_xi/1
  ug_abc_pu/1 -> Demux/1
  Demux/1 -> filter_and_transformation/1(ug_a)
  Demux/2 -> filter_and_transformation/2(ug_b)
  Demux/3 -> filter_and_transformation/3(ug_c)
  filter_and_transformation/1(ug_alpha) -> Math Function/1, sequences/1(u_grid_alpha)
  filter_and_transformation/2(ug_beta) -> Math Function1/1, sequences/2(u_grid_beta)
  Math Function/1 -> Sum/1
  Math Function1/1 -> Sum/2
  Sum/1 -> Saturation/1
  Reciprocal Sqrt/1 -> [Vgrid_unorm_fht]
  Saturation/1 -> Reciprocal Sqrt/1

== system single_phase_ttype_inverter/afe/AFE_control/afe_control/grid_voltage_phase_lock_loops/FHT-PLL/pll_stageB ==
  u_grid_pos_xi : Inport
  u_grid_pos_eta : Inport  Port=2
  Constant4 : Constant  Value=grid_emu.omega_grid_nom
  Gain : Gain  Gain=-1
  Product : Product  RndMeth=Zero
  Product1 : Product  RndMeth=Zero
  Product2 : Product  RndMeth=Zero
  Sum3 : Sum  SaturateOnIntegerOverflow=on
  Sum4 : Sum  SaturateOnIntegerOverflow=on
  Sum5 : Sum  Inputs=++|
  Terminator : Terminator
  Unit Delay1 : UnitDelay  SampleTime=-1
  Unit Delay2 : UnitDelay  SampleTime=-1
  Unit Delay4 : UnitDelay  SampleTime=-1
  bounder1 : MATLAB Function  TreatAsAtomicUnit=on
  double_integrator_observer : Subsystem
  kp : Gain  Gain=afe_ctrl.pll_i1_fht*glb_time.ts_afe  SaturateOnIntegerOverflow=on  OutDataTypeStr=Inherit: Same as input  ParamDataTypeStr=Inherit: Same as input
  kp1 : Gain  Gain=afe_ctrl.pll_p_fht  SaturateOnIntegerOverflow=on  OutDataTypeStr=Inherit: Same as input  ParamDataTypeStr=Inherit: Same as input
  kp2 : Gain  Gain=glb_time.ts_afe  SaturateOnIntegerOverflow=on  OutDataTypeStr=Inherit: Same as input  ParamDataTypeStr=Inherit: Same as input
  kp3 : Gain  Gain=1/grid_emu.omega_grid_nom  SaturateOnIntegerOverflow=on  OutDataTypeStr=Inherit: Same as input  ParamDataTypeStr=Inherit: Same as input
  gamma_grid_ddsrf_pll : Outport  VectorParamsAs1DForOutWhenUnconnected=off
  omega_grid_ddsrf_pll : Outport  Port=2  VectorParamsAs1DForOutWhenUnconnected=off
  wires:
  Gain/1 -> kp/1, kp1/1
  Product1/1 -> Gain/1
  kp3/1 -> omega_grid_ddsrf_pll/1
  Product/1 -> Terminator/1
  double_integrator_observer/1(omega_hat) -> kp3/1
  Unit Delay4/1 -> Sum3/2
  Sum4/1 -> bounder1/1(u)
  Unit Delay1/1 -> Sum4/2
  Sum3/1 -> Sum5/2, Unit Delay4/1  "i1"
  kp2/1 -> Sum4/1
  Constant4/1 -> Product2/2
  [Vgrid_unorm_fht] -> Product/2, Product1/2
  kp/1 -> Sum3/1
  Sum5/1 -> Product2/1
  bounder1/1(y) -> Unit Delay2/1, Unit Delay1/1
  u_grid_pos_xi/1 -> Product/1
  u_grid_pos_eta/1 -> Product1/1
  Product2/1 -> kp2/1
  kp1/1 -> Sum5/1
  Unit Delay2/1 -> double_integrator_observer/1(theta), gamma_grid_ddsrf_pll/1

== system single_phase_ttype_inverter/afe/AFE_control/afe_control/grid_voltage_phase_lock_loops/dq_pll/pll_stageA ==
  phase_grid : Inport
  ug_abc : Inport  Port=2
  Demux : Demux  Outputs=3
  Math Function : Math  Operator=magnitude^2  SignedPower=on
  Math Function1 : Math  Operator=magnitude^2  SignedPower=on
  Reciprocal Sqrt : Sqrt  Operator=rSqrt
  Saturation : Saturate  UpperLimit=inf  LowerLimit=0.02
  Sum : Sum  Inputs=|++
  mormalization_and_transformation : Subsystem
  sequences : Subsystem
  u_grid_pos_xi : Outport  VectorParamsAs1DForOutWhenUnconnected=off
  u_grid_pos_eta : Outport  Port=2  VectorParamsAs1DForOutWhenUnconnected=off
  tag scope: Vgrid_unorm_dqpll=scoped
  wires:
  ug_abc/1 -> Demux/1
  Demux/1 -> mormalization_and_transformation/1(ug_a)
  Demux/2 -> mormalization_and_transformation/2(ug_b)
  Demux/3 -> mormalization_and_transformation/3(ug_c)
  phase_grid/1 -> sequences/3(gamma_grid)
  sequences/1(u_grid_pos_xi) -> u_grid_pos_xi/1
  sequences/2(u_grid_pos_eta) -> u_grid_pos_eta/1
  Math Function1/1 -> Sum/2
  mormalization_and_transformation/1(ug_alpha) -> Math Function/1, sequences/1(u_grid_alpha)
  mormalization_and_transformation/2(ug_beta) -> Math Function1/1, sequences/2(u_grid_beta)
  Reciprocal Sqrt/1 -> [Vgrid_unorm_dqpll]
  Sum/1 -> Saturation/1
  Math Function/1 -> Sum/1
  Saturation/1 -> Reciprocal Sqrt/1

== system single_phase_ttype_inverter/afe/AFE_control/afe_control/grid_voltage_phase_lock_loops/dq_pll/pll_stageB ==
  u_grid_pos_xi : Inport
  u_grid_pos_eta : Inport  Port=2
  -2<x<2 : Saturate  UpperLimit=2  LowerLimit=-2
  Constant4 : Constant  Value=grid_emu.omega_grid_nom
  Gain : Gain  Gain=1/grid_emu.omega_grid_nom
  Product1 : Product  RndMeth=Zero
  Product2 : Product  RndMeth=Zero
  Sum3 : Sum  SaturateOnIntegerOverflow=on
  Sum4 : Sum  SaturateOnIntegerOverflow=on
  Sum5 : Sum  Inputs=++|
  Terminator : Terminator
  Unit Delay1 : UnitDelay  SampleTime=-1
  Unit Delay2 : UnitDelay  SampleTime=-1
  Unit Delay4 : UnitDelay  SampleTime=-1
  bounder1 : MATLAB Function  TreatAsAtomicUnit=on
  double_integrator_observer : Subsystem
  kp : Gain  Gain=afe_ctrl.pll_i1*glb_time.ts_afe  SaturateOnIntegerOverflow=on  OutDataTypeStr=Inherit: Same as input  ParamDataTypeStr=Inherit: Same as input
  kp2 : Gain  Gain=glb_time.ts_afe  SaturateOnIntegerOverflow=on  OutDataTypeStr=Inherit: Same as input  ParamDataTypeStr=Inherit: Same as input
  scheduled-p-gain : Subsystem
      settings: PortSchema="{\"entries\":[{\"content\":{\"sides\":[{\"content\":{},\"type\":\"ConnectorPlacement.EquallySpacedRectSide\",\"uuid\":\"88e64df2-a299-4c1b-9bac-7a615cd04a00\"},{\"content\":{\"side\":\"RIGHT\"},\"type\":\"ConnectorPlacement.EquallySpacedRectSide\",\"uuid\":\"ef1d7318-b0e2-4e96-bf99-c42bb4ec5202\"},{\"content\":{\"connectorIds\":[\"In1\"],\"side\":\"TOP\"},\"type\":\"ConnectorPlacement.EquallySpacedRectSide\",\"uuid\":\"96582c59-f6c8-40f1-b3cf-394cc239c4b2\"},{\"content\":{\"connectorIds\":[\"Out1\"],\"side\":\"BOTTOM\"},\"type\":\"ConnectorPlacement.EquallySpacedRectSide\",\"uuid\":\"9ac5cd0d-958f-4b67-b4ea-90856a0aa038\"}]},\"type\":\"ConnectorPlacement.EquallySpacedConnector\",\"uuid\":\"ca37db80-6b94-4315-bd9c-66307567cd1f\"}],\"packageUris\":[\"http://schema.mathworks.com/mf0/Connector/R2020b\"],\"version\":\"1.0\"}"
  phase_grid_pll : Outport  VectorParamsAs1DForOutWhenUnconnected=off
  omega_grid_pu_pll : Outport  Port=2  VectorParamsAs1DForOutWhenUnconnected=off
  wires:
  Unit Delay4/1 -> Sum3/2
  Sum3/1 -> -2<x<2/1
  Sum4/1 -> bounder1/1(u)
  Unit Delay1/1 -> Sum4/2
  -2<x<2/1 -> Sum5/2, Unit Delay4/1  "i1"
  kp2/1 -> Sum4/1
  Constant4/1 -> Product2/2
  [Vgrid_unorm_dqpll] -> Product1/2
  kp/1 -> Sum3/1
  Sum5/1 -> Product2/1
  bounder1/1(y) -> Unit Delay1/1, Unit Delay2/1
  u_grid_pos_eta/1 -> Product1/1
  Product2/1 -> kp2/1
  Product1/1 -> scheduled-p-gain/1(In1), kp/1
  scheduled-p-gain/1(Out2) -> Sum5/1
  Unit Delay2/1 -> double_integrator_observer/1(phase), phase_grid_pll/1
  double_integrator_observer/1(omega_hat) -> Gain/1
  Gain/1 -> omega_grid_pu_pll/1
  u_grid_pos_xi/1 -> Terminator/1
